simulink model "RobustFormationControl_IntegerModel_under_Dis"  (R2023a)
settings: Solver=ode3  StartTime=0.0  StopTime=30  FixedStep=0.0001  RelTol=1e-3
InitFcn:
  | % % Parameters for the fractional order NTFSMC:
  | % Sliding Surface " Sx, Sy, and Sz ":
  | %------------------------
  | % 10
  | % 10
  | cx = 2*[4 4 4];
  | cxx = 1*[0.01 0.01 0.01];
  | 
  | cx1 = cx(1);
  | cy1 = cx(2);
  | cz1 = cx(3);
  | 
  | cx2 = cxx(1);
  | cy2 = cxx(2);
  | cz2 = cxx(3);
  | 
  | alpha1 = [0.6 0.6 0.6];
  | alpha2 = [0.1 0.1 0.1];
  | 
  | gammaX = [3 3 3];
  | gx  = gammaX(1);
  | gy = gammaX(2);
  | gz = gammaX(3);
  | 
  | p = 10;
  | q = 10;
  | 
  | % Sliding Surface " S_Phi , S_Theta, and  S_Psi":
  | %------------------------
  | cP = 2*[4 4 4];
  | cPP = 1*[0.01 0.01 0.01 0.01];
  | 
  | cPhi1 = cP(1);
  | cTheta1 = cP(2);
  | cPsi1 = cP(3);
  | 
  | cPhi2 = cPP(1);
  | cTheta2 = cPP(2);
  | cPsi2 = cPP(3);
  | gammaP = [3 3 3];
  | 
  | %=========================
  | %=========================
  | SigmaX = 1*[0.01 0.01 0.01];
  | SigmaXX =1*[1 1 1];
  | 
  | Sigma1X = SigmaX(1);
  | Sigma1Y = SigmaX(2);
  | Sigma1Z = SigmaX(3);
  | %-----
  | Sigma2X = SigmaXX(1);
  | Sigma2Y = SigmaXX(2);
  | Sigma2Z = SigmaXX(3);
  | 
  | 
  | SigmaP = 1*[0.01 0.01 0.01];
  | SigmaPP =1*[1 1 1];
  | 
  | Sigma1Phi   = SigmaP(1);
  | Sigma1Theta = SigmaP(2);
  | ... (+80 lines)
values from neighbouring files (symbols this model uses):
  a1 = (Iyy - Izz)/Ixx    (= -0.812397034596)    [init_quadrotor_params.m]
  a2 = (Izz - Ixx)/Iyy    (= 0.812397034596)    [init_quadrotor_params.m]
  a3 = (Ixx - Iyy)/Izz    (= 0)    [init_quadrotor_params.m]
  a4 = - Ktx/m    (= -0.00114547325103)    [init_quadrotor_params.m]
  a5 = - Kty/m    (= -0.00114547325103)    [init_quadrotor_params.m]
  a6 = - Ktz/m    (= -0.00130740740741)    [init_quadrotor_params.m]
  b = 2.980e-5    (= 2.98e-05)    [init_quadrotor_params.m]
  b1 = - Jr/Ixx    (= -0.00584534596376)    [init_quadrotor_params.m]
  b2 = Jr/Iyy    (= 0.00584534596376)    [init_quadrotor_params.m]
  b3 = - Kfz/Izz    (= -0.0721963413248)    [init_quadrotor_params.m]
  b4 = 1/m    (= 2.05761316872)    [init_quadrotor_params.m]
  b5 = 1/m    (= 2.05761316872)    [init_quadrotor_params.m]
  b6 = 1/m    (= 2.05761316872)    [init_quadrotor_params.m]
  c1 = - Kfx/Ixx    (= -0.114641680395)    [init_quadrotor_params.m]
  c2 = - Kfy/Iyy    (= -0.114641680395)    [init_quadrotor_params.m]
  c3 = 1/Izz    (= 113.62345188)    [init_quadrotor_params.m]
  d = 1.12e-06    [init_quadrotor_params.m]
  d1 = L/Ixx    (= 46.334431631)    [init_quadrotor_params.m]
  d2 = L/Iyy    (= 46.334431631)    [init_quadrotor_params.m]
  g = 9.81    [init_quadrotor_params.m]
  Ixx = 4.856e-3    (= 0.004856)    [init_quadrotor_params.m]
  Iyy = 4.856e-3    (= 0.004856)    [init_quadrotor_params.m]
  Izz = 8.801e-3    (= 0.008801)    [init_quadrotor_params.m]
  Jr = 2.8385e-5    (= 2.8385e-05)    [init_quadrotor_params.m]
  Kfx = 5.567e-4    (= 0.0005567)    [init_quadrotor_params.m]
  Kfy = 5.567e-4    (= 0.0005567)    [init_quadrotor_params.m]
  Kfz = 6.354e-4    (= 0.0006354)    [init_quadrotor_params.m]
  Ktx = 5.5670e-4    (= 0.0005567)    [init_quadrotor_params.m]
  Kty = 5.5670e-4    (= 0.0005567)    [init_quadrotor_params.m]
  Ktz = 6.3540e-4    (= 0.0006354)    [init_quadrotor_params.m]
  L = 0.225    [init_quadrotor_params.m]
  m = 0.486    [init_quadrotor_params.m]
libraries: fod x120, eeStairGenerator x5
(part 6 of 9)

== system RobustFormationControl_IntegerModel_under_Dis/Integer Leader and four followers/Follower 1 System/Follower 1 Quadrotor Model/Control Module1/Subsystem5/Subsystem ==
  x5 : Inport
  xd5 : Inport  Port=2
  x6 : Inport  Port=3
  xd6 : Inport  Port=4
  S4 : Inport  Port=5
  Constant : Constant  Value=p/q
  Constant1 : Constant  Value=gammaP(3)-1
  Divide : Product  Inputs=**  RndMeth=Zero  SaturateOnIntegerOverflow=on
  Fractional derivative : fod/Fractional derivative  gam=alpha1(3)  ww=[0.001; 1000]  n=5  nFod=off
      settings: SourceProductName=FOMCON Toolbox
  Fractional integrator1 : fod/Fractional integrator  gam=alpha2(2)  ww=[0.001; 1000]  n=5  nFod=off
      settings: SourceProductName=FOMCON Toolbox
  Gain : Gain  Gain=cPsi1
  Gain1 : Gain  Gain=cPsi2
  Gain2 : Gain  Gain=gammaP(3)
  Gain3 : Gain  Gain=Sigma1Psi
  Gain4 : Gain  Gain=Sigma2Psi
  Power : Math  Operator=pow
  Power1 : Math  Operator=pow
  Sign : Signum
  Sum : Sum
  Sum1 : Sum  Inputs=+-
  Sum2 : Sum  Inputs=---
  Sum3 : Sum  Inputs=+-
  D2 : Outport  VectorParamsAs1DForOutWhenUnconnected=off
  wires:
  xd6/1 -> Sum1/2
  xd5/1 -> Sum3/2
  x5/1 -> Sum3/1
  x6/1 -> Sum1/1
  Sum3/1 -> Power1/1, Power/1
  Constant/1 -> Power/2
  Power/1 -> Gain/1
  Gain/1 -> Fractional derivative/1
  Constant1/1 -> Power1/2
  Power1/1 -> Divide/2
  Divide/1 -> Gain1/1
  Gain1/1 -> Gain2/1
  Sum1/1 -> Divide/1
  Gain2/1 -> Fractional integrator1/1
  S4/1 -> Gain4/1, Sign/1
  Sign/1 -> Gain3/1
  Gain3/1 -> Sum/1
  Gain4/1 -> Sum/2
  Sum/1 -> Sum2/3
  Fractional derivative/1 -> Sum2/1
  Fractional integrator1/1 -> Sum2/2
  Sum2/1 -> D2/1

== system RobustFormationControl_IntegerModel_under_Dis/Integer Leader and four followers/Follower 1 System/Follower 1 Quadrotor Model/Control Module1/Subsystem5/Subsystem1 ==
  x4 : Inport
  x6 : Inport  Port=2
  x2 : Inport  Port=3
  xd6 : Inport  Port=4
  Gain : Gain  Gain=a3
  Gain6 : Gain  Gain=b3
  Math Function : Math  Operator=square  SignedPower=on
  Product1 : Product
  Sum1 : Sum  Inputs=--+
  D1 : Outport
  wires:
  x6/1 -> Math Function/1
  Product1/1 -> Gain/1
  xd6/1 -> Sum1/3
  Gain6/1 -> Sum1/2  "c1 x2^2"
  Math Function/1 -> Gain6/1  "x2^2"
  x2/1 -> Product1/1
  Gain/1 -> Sum1/1  "a1 x4 x6"
  x4/1 -> Product1/2
  Sum1/1 -> D1/1

== system RobustFormationControl_IntegerModel_under_Dis/Integer Leader and four followers/Follower 1 System/Follower 1 Quadrotor Model/Control Module1/Subsystem5/Subsystem2 ==
  x5 : Inport
  xd5 : Inport  Port=2
  x6 : Inport  Port=3
  xd6 : Inport  Port=4
  S6 : Inport  Port=5
  Abs : Abs  SaturateOnIntegerOverflow=off
  Divide{,1..4} (5 alike) : Product  Inputs=**  RndMeth=Zero  SaturateOnIntegerOverflow=on
  Gain : Gain  Gain=q0
  Gain1 : Gain  Gain=q1
  Gain2 : Gain  Gain=q2
  Integrator : Integrator
  Integrator1 : Integrator
  Integrator2 : Integrator
  Sign : Signum
  Sum1 : Sum  Inputs=+-
  Sum2 : Sum  Inputs=----
  Sum3 : Sum  Inputs=+-
  w : Constant  Value=w
  D3 : Outport  VectorParamsAs1DForOutWhenUnconnected=off
  wires:
  xd6/1 -> Sum1/2
  xd5/1 -> Sum3/2
  x5/1 -> Sum3/1
  x6/1 -> Sum1/1
  S6/1 -> [S6], Abs/1
  Sum1/1 -> [e2]
  Sum3/1 -> [e1]
  Gain/1 -> Integrator/1
  Integrator/1 -> Sum2/1  "B0"
  [e1] -> Divide/2
  Gain1/1 -> Integrator1/1
  Divide/1 -> Gain1/1
  Divide1/1 -> Gain2/1
  Gain2/1 -> Integrator2/1
  [e2] -> Divide1/2
  Abs/1 -> Divide1/1, Divide/1, Gain/1
  Integrator1/1 -> Divide3/2  "B1"
  w/1 -> Sum2/4
  Sign/1 -> Divide2/2
  [S6] -> Sign/1
  Divide2/1 -> D3/1
  [e1] -> Divide3/1
  [e2] -> Divide4/1
  Integrator2/1 -> Divide4/2  "B2"
  Divide3/1 -> Sum2/2
  Divide4/1 -> Sum2/3
  Sum2/1 -> Divide2/1

== system RobustFormationControl_IntegerModel_under_Dis/Integer Leader and four followers/Follower 1 System/Follower 1 Quadrotor Model/Control Module1/Subsystem6/Subsystem3 ==
  xL : Inport
  x7 : Inport  Port=2
  x8 : Inport  Port=3
  dX : Inport  Port=4
  S8 : Inport  Port=5
  Constant : Constant  Value=p/q
  Constant1 : Constant  Value=gx-1
  Derivative : Derivative
  Derivative1 : Derivative
  Divide : Product  Inputs=**  RndMeth=Zero  SaturateOnIntegerOverflow=on
  Fractional derivative : fod/Fractional derivative  gam=alpha1(1)  ww=[0.001; 1000]  n=5  nFod=off
      settings: SourceProductName=FOMCON Toolbox
  Fractional integrator1 : fod/Fractional integrator  gam=alpha2(1)  ww=[0.001; 1000]  n=5  nFod=off
      settings: SourceProductName=FOMCON Toolbox
  Gain : Gain  Gain=cx1
  Gain1 : Gain  Gain=cx2
  Gain2 : Gain  Gain=gx
  Gain3 : Gain  Gain=Sigma1X
  Gain4 : Gain  Gain=Sigma2X
  Power : Math  Operator=pow
  Power1 : Math  Operator=pow
  Sign : Signum
  Sum : Sum
  Sum1 : Sum  Inputs=+--
  Sum2 : Sum  Inputs=+++
  Sum3 : Sum  Inputs=+--
  D2 : Outport  VectorParamsAs1DForOutWhenUnconnected=off
  wires:
  Sum3/1 -> Power1/1, Power/1
  Constant/1 -> Power/2
  Power/1 -> Gain/1
  Gain/1 -> Fractional derivative/1
  Constant1/1 -> Power1/2
  Power1/1 -> Divide/2
  Divide/1 -> Gain1/1
  Gain1/1 -> Gain2/1
  Sum1/1 -> Divide/1
  Gain2/1 -> Fractional integrator1/1
  S8/1 -> Gain4/1, Sign/1
  Sign/1 -> Gain3/1
  Gain3/1 -> Sum/1
  Gain4/1 -> Sum/2
  Sum/1 -> Sum2/3
  Fractional derivative/1 -> Sum2/1
  Fractional integrator1/1 -> Sum2/2
  Sum2/1 -> D2/1
  xL/1 -> Sum3/1, Derivative/1
  Derivative/1 -> Sum1/1
  x8/1 -> Sum1/2
  dX/1 -> Sum3/3, Derivative1/1
  Derivative1/1 -> Sum1/3
  x7/1 -> Sum3/2

== system RobustFormationControl_IntegerModel_under_Dis/Integer Leader and four followers/Follower 1 System/Follower 1 Quadrotor Model/Control Module1/Subsystem6/Subsystem4 ==
  x8 : Inport
  xL : Inport  Port=2
  dX : Inport  Port=3
  Derivative{,1..3} (4 alike) : Derivative
  Divide2 : Product  Inputs=**  RndMeth=Zero  SaturateOnIntegerOverflow=on
  Gain1 : Gain  Commented=on  Gain=a6
  Sum : Sum  Inputs=-+-
  D1 : Outport
  wires:
  Sum/1 -> D1/1
  x8/1 -> Divide2/2
  Divide2/1 -> Sum/1
  [a4D] -> Divide2/1
  Derivative/1 -> Derivative1/1
  xL/1 -> Derivative/1
  Derivative3/1 -> Sum/3
  Derivative2/1 -> Derivative3/1
  dX/1 -> Derivative2/1
  Derivative1/1 -> Sum/2

== system RobustFormationControl_IntegerModel_under_Dis/Integer Leader and four followers/Follower 1 System/Follower 1 Quadrotor Model/Control Module1/Subsystem6/Subsystem5 ==
  xL : Inport
  x7 : Inport  Port=2
  x8 : Inport  Port=3
  dX : Inport  Port=4
  S8 : Inport  Port=5
  Abs : Abs  SaturateOnIntegerOverflow=off
  Derivative : Derivative
  Derivative1 : Derivative
  Divide{,1..4} (5 alike) : Product  Inputs=**  RndMeth=Zero  SaturateOnIntegerOverflow=on
  Gain : Gain  Gain=q0
  Gain1 : Gain  Gain=q1
  Gain2 : Gain  Gain=q2
  Integrator : Integrator
  Integrator1 : Integrator
  Integrator2 : Integrator
  Mux : Mux  Inputs=3
  Sign : Signum
  Sum2 : Sum  Inputs=++++
  Sum4 : Sum  Inputs=+--
  Sum5 : Sum  Inputs=+--
  To Workspace : ToWorkspace  VariableName=BxF1  SampleTime=-1
  w : Constant  Value=w
  D3 : Outport  VectorParamsAs1DForOutWhenUnconnected=off
  wires:
  S8/1 -> [S8], Abs/1
  Gain/1 -> Integrator/1
  [e1] -> Divide/2
  Gain1/1 -> Integrator1/1
  Divide/1 -> Gain1/1
  Divide1/1 -> Gain2/1
  Gain2/1 -> Integrator2/1
  [e2] -> Divide1/2
  Abs/1 -> Divide1/1, Divide/1, Gain/1
  Integrator1/1 -> Divide3/2  "B1"
  w/1 -> Sum2/4
  Sign/1 -> Divide2/2
  [S8] -> Sign/1
  Divide2/1 -> D3/1
  [e1] -> Divide3/1
  [e2] -> Divide4/1
  Integrator2/1 -> Divide4/2  "B2"
  Sum2/1 -> Divide2/1
  Derivative1/1 -> Sum4/3
  Derivative/1 -> Sum4/1
  Sum4/1 -> [e2]
  Sum5/1 -> [e1]
  xL/1 -> Sum5/1, Derivative/1
  x8/1 -> Sum4/2
  dX/1 -> Sum5/3, Derivative1/1
  x7/1 -> Sum5/2
  Integrator/1 -> Mux/1, Sum2/1  "B0"
  Divide3/1 -> Mux/2, Sum2/2
  Divide4/1 -> Mux/3, Sum2/3
  Mux/1 -> To Workspace/1

== system RobustFormationControl_IntegerModel_under_Dis/Integer Leader and four followers/Follower 1 System/Follower 1 Quadrotor Model/Control Module1/Subsystem8/Subsystem ==
  x3 : Inport
  xd3 : Inport  Port=2
  x4 : Inport  Port=3
  xd4 : Inport  Port=4
  S4 : Inport  Port=5
  Constant : Constant  Value=p/q
  Constant1 : Constant  Value=gammaP(2)-1
  Divide : Product  Inputs=**  RndMeth=Zero  SaturateOnIntegerOverflow=on
  Fractional derivative : fod/Fractional derivative  gam=alpha1(2)  ww=[0.001; 1000]  n=5  nFod=off
      settings: SourceProductName=FOMCON Toolbox
  Fractional integrator1 : fod/Fractional integrator  gam=alpha2(2)  ww=[0.001; 1000]  n=5  nFod=off
      settings: SourceProductName=FOMCON Toolbox
  Gain : Gain  Gain=cTheta1
  Gain1 : Gain  Gain=cTheta2
  Gain2 : Gain  Gain=gammaP(2)
  Gain3 : Gain  Gain=Sigma1Theta
  Gain4 : Gain  Gain=Sigma2Theta
  Power : Math  Operator=pow
  Power1 : Math  Operator=pow
  Sign : Signum
  Sum : Sum
  Sum1 : Sum  Inputs=+-
  Sum2 : Sum  Inputs=---
  Sum3 : Sum  Inputs=+-
  D2 : Outport  VectorParamsAs1DForOutWhenUnconnected=off
  wires:
  xd4/1 -> Sum1/2
  xd3/1 -> Sum3/2
  x3/1 -> Sum3/1
  x4/1 -> Sum1/1
  Sum3/1 -> Power1/1, Power/1
  Constant/1 -> Power/2
  Power/1 -> Gain/1
  Gain/1 -> Fractional derivative/1
  Constant1/1 -> Power1/2
  Power1/1 -> Divide/2
  Divide/1 -> Gain1/1
  Gain1/1 -> Gain2/1
  Sum1/1 -> Divide/1
  Gain2/1 -> Fractional integrator1/1
  S4/1 -> Gain4/1, Sign/1
  Sign/1 -> Gain3/1
  Gain3/1 -> Sum/1
  Gain4/1 -> Sum/2
  Sum/1 -> Sum2/3
  Fractional derivative/1 -> Sum2/1
  Fractional integrator1/1 -> Sum2/2
  Sum2/1 -> D2/1

== system RobustFormationControl_IntegerModel_under_Dis/Integer Leader and four followers/Follower 1 System/Follower 1 Quadrotor Model/Control Module1/Subsystem8/Subsystem1 ==
  x4 : Inport
  x6 : Inport  Port=2
  x2 : Inport  Port=3
  Omega : Inport  Port=4
  xd4 : Inport  Port=5
  Gain1 : Gain  Gain=a2
  Gain2 : Gain  Gain=c2
  Gain3 : Gain  Gain=b2
  Math Function1 : Math  Operator=square  SignedPower=on
  Product2 : Product
  Product4 : Product
  Sum3 : Sum  Inputs=---+
  D1 : Outport
  wires:
  x6/1 -> Product2/2
  Gain1/1 -> Sum3/1  "a1 x4 x6"
  Sum3/1 -> D1/1
  Math Function1/1 -> Gain2/1  "x2^2"
  x2/1 -> Product4/1, Product2/1
  x4/1 -> Math Function1/1
  xd4/1 -> Sum3/4
  Product4/1 -> Gain3/1
  Omega/1 -> Product4/2
  Product2/1 -> Gain1/1
  Gain3/1 -> Sum3/3
  Gain2/1 -> Sum3/2  "c1 x2^2"

== system RobustFormationControl_IntegerModel_under_Dis/Integer Leader and four followers/Follower 1 System/Follower 1 Quadrotor Model/Control Module1/Subsystem8/Subsystem2 ==
  x3 : Inport
  xd3 : Inport  Port=2
  x4 : Inport  Port=3
  xd4 : Inport  Port=4
  S4 : Inport  Port=5
  Abs : Abs  SaturateOnIntegerOverflow=off
  Divide{,1..4} (5 alike) : Product  Inputs=**  RndMeth=Zero  SaturateOnIntegerOverflow=on
  Gain : Gain  Gain=q0
  Gain1 : Gain  Gain=q1
  Gain2 : Gain  Gain=q2
  Integrator : Integrator
  Integrator1 : Integrator
  Integrator2 : Integrator
  Sign : Signum
  Sum1 : Sum  Inputs=+-
  Sum2 : Sum  Inputs=----
  Sum3 : Sum  Inputs=+-
  w : Constant  Value=w
  D3 : Outport  VectorParamsAs1DForOutWhenUnconnected=off
  wires:
  xd4/1 -> Sum1/2
  xd3/1 -> Sum3/2
  x3/1 -> Sum3/1
  x4/1 -> Sum1/1
  S4/1 -> [S4], Abs/1
  Sum1/1 -> [e2]
  Sum3/1 -> [e1]
  Gain/1 -> Integrator/1
  Integrator/1 -> Sum2/1  "B0"
  [e1] -> Divide/2
  Gain1/1 -> Integrator1/1
  Divide/1 -> Gain1/1
  Divide1/1 -> Gain2/1
  Gain2/1 -> Integrator2/1
  [e2] -> Divide1/2
  Abs/1 -> Divide1/1, Divide/1, Gain/1
  Integrator1/1 -> Divide3/2  "B1"
  w/1 -> Sum2/4
  Sign/1 -> Divide2/2
  [S4] -> Sign/1
  Divide2/1 -> D3/1
  [e1] -> Divide3/1
  [e2] -> Divide4/1
  Integrator2/1 -> Divide4/2  "B2"
  Divide3/1 -> Sum2/2
  Divide4/1 -> Sum2/3
  Sum2/1 -> Divide2/1

== system RobustFormationControl_IntegerModel_under_Dis/Integer Leader and four followers/Follower 1 System/Follower 1 Quadrotor Model/Quadrotor Dynamic System/Rotational System/Equation1 ==
  x4 : Inport
  x6 : Inport  Port=2
  U2 : Inport  Port=3
  Omega : Inport  Port=4
  Gain : Gain  Gain=a1
  Gain1 : Gain  Gain=c1
  Gain2 : Gain  Gain=b1
  Gain3 : Gain  Gain=d1
  Integrator : Integrator
  Integrator1 : Integrator
  Math Function : Math  Operator=square  SignedPower=on
  Product : Product
  Product1 : Product
  Sum : Sum  Inputs=|++++
  x1 = Phi : Outport  VectorParamsAs1DForOutWhenUnconnected=off
  x2 : Outport  Port=2  VectorParamsAs1DForOutWhenUnconnected=off
  wires:
  Math Function/1 -> Gain1/1  "x2^2"
  x4/1 -> Product1/1, Product/1
  Integrator/1 -> Math Function/1, x2/1, Integrator1/1
  U2/1 -> Gain3/1
  Gain2/1 -> Sum/3
  Gain3/1 -> Sum/4
  Gain/1 -> Sum/1  "a1 x4 x6"
  Product1/1 -> Gain2/1
  Gain1/1 -> Sum/2  "c1 x2^2"
  Integrator1/1 -> x1 = Phi/1
  Product/1 -> Gain/1
  x6/1 -> Product/2
  Sum/1 -> Integrator/1
  Omega/1 -> Product1/2

== system RobustFormationControl_IntegerModel_under_Dis/Integer Leader and four followers/Follower 1 System/Follower 1 Quadrotor Model/Quadrotor Dynamic System/Rotational System/Equation2 ==
  x2 : Inport
  x6 : Inport  Port=2
  U3 : Inport  Port=3
  Omega : Inport  Port=4
  Gain : Gain  Gain=a2
  Gain1 : Gain  Gain=c2
  Gain2 : Gain  Gain=b2
  Gain3 : Gain  Gain=d2
  Integrator : Integrator
  Integrator1 : Integrator
  Math Function : Math  Operator=square  SignedPower=on
  Product : Product
  Product1 : Product
  Sum : Sum  Inputs=|++++
  x3 =Theta : Outport  VectorParamsAs1DForOutWhenUnconnected=off
  x4 : Outport  Port=2  VectorParamsAs1DForOutWhenUnconnected=off
  wires:
  Math Function/1 -> Gain1/1  "x4^2"
  x2/1 -> Product1/1, Product/1
  Integrator/1 -> Math Function/1, x4/1, Integrator1/1
  U3/1 -> Gain3/1
  Gain2/1 -> Sum/3
  Gain3/1 -> Sum/4
  Gain/1 -> Sum/1  "a2 x2 x6"
  Product1/1 -> Gain2/1
  Gain1/1 -> Sum/2  "c2 x2^2"
  Integrator1/1 -> x3 =Theta/1
  Product/1 -> Gain/1
  x6/1 -> Product/2
  Sum/1 -> Integrator/1
  Omega/1 -> Product1/2

== system RobustFormationControl_IntegerModel_under_Dis/Integer Leader and four followers/Follower 1 System/Follower 1 Quadrotor Model/Quadrotor Dynamic System/Rotational System/Equation3 ==
  x2 : Inport
  x4 : Inport  Port=2
  U4 : Inport  Port=3
  Gain : Gain  Gain=a3
  Gain1 : Gain  Gain=b3
  Gain3 : Gain  Gain=c3
  Integrator : Integrator
  Integrator1 : Integrator
  Math Function : Math  Operator=square  SignedPower=on
  Product : Product
  Sum : Sum  Inputs=|+++
  x5 =Psi : Outport  VectorParamsAs1DForOutWhenUnconnected=off
  x6 : Outport  Port=2  VectorParamsAs1DForOutWhenUnconnected=off
  wires:
  Math Function/1 -> Gain1/1  "x6^2"
  x2/1 -> Product/1
  Integrator/1 -> Math Function/1, x6/1, Integrator1/1
  U4/1 -> Gain3/1
  Gain3/1 -> Sum/3
  Gain/1 -> Sum/1  "a3 x2 x4"
  Gain1/1 -> Sum/2  "b3 x6^2"
  Integrator1/1 -> x5 =Psi/1
  Product/1 -> Gain/1
  x4/1 -> Product/2
  Sum/1 -> Integrator/1

== system RobustFormationControl_IntegerModel_under_Dis/Integer Leader and four followers/Follower 1 System/Follower 1 Quadrotor Model/Quadrotor Dynamic System/Translational System/Equation4 ==
  U1 : Inport
  Ux : Inport  Port=2
  Gain : Gain  Gain=1/m
  Gain1 : Gain  Gain=a4
  Integrator : Integrator
  Integrator1 : Integrator  InitialCondition=2
  Product : Product
  Sum : Sum  Inputs=|++
  x7 = x : Outport  VectorParamsAs1DForOutWhenUnconnected=off
  x8 = xdot : Outport  Port=2  VectorParamsAs1DForOutWhenUnconnected=off
  wires:
  Integrator/1 -> Gain1/1, x8 = xdot/1, Integrator1/1
  U1/1 -> Product/1
  Gain/1 -> Sum/1  "U1 Ux / m"
  Gain1/1 -> Sum/2  "a4 x8"
  Integrator1/1 -> x7 = x/1
  Product/1 -> Gain/1
  Ux/1 -> Product/2
  Sum/1 -> Integrator/1

== system RobustFormationControl_IntegerModel_under_Dis/Integer Leader and four followers/Follower 1 System/Follower 1 Quadrotor Model/Quadrotor Dynamic System/Translational System/Equation5 ==
  U1 : Inport
  Uy : Inport  Port=2
  Gain : Gain  Gain=1/m
  Gain1 : Gain  Gain=a5
  Integrator : Integrator
  Integrator1 : Integrator  InitialCondition=-2
  Product : Product
  Sum : Sum  Inputs=|++
  x9 = y : Outport  VectorParamsAs1DForOutWhenUnconnected=off
  x10 = ydot : Outport  Port=2  VectorParamsAs1DForOutWhenUnconnected=off
  wires:
  Integrator/1 -> x10 = ydot/1, Integrator1/1, Gain1/1
  U1/1 -> Product/1
  Gain/1 -> Sum/1  "U1 Ux / m"
  Gain1/1 -> Sum/2  "a4 x10"
  Integrator1/1 -> x9 = y/1
  Product/1 -> Gain/1
  Uy/1 -> Product/2
  Sum/1 -> Integrator/1

== system RobustFormationControl_IntegerModel_under_Dis/Integer Leader and four followers/Follower 1 System/Follower 1 Quadrotor Model/Quadrotor Dynamic System/Translational System/Equation6 ==
  U1 : Inport
  x1 : Inport  Port=2
  x3 : Inport  Port=3
  Constant : Constant  Value=g
  Gain : Gain  Gain=1/m
  Gain1 : Gain  Gain=a6
  Integrator : Integrator
  Integrator1 : Integrator
  Product : Product
  Product1 : Product
  Sum : Sum  Inputs=|++-
  Trigonometric Function : Trigonometry  Operator=cos
  Trigonometric Function1 : Trigonometry  Operator=cos
  x11 = z : Outport  VectorParamsAs1DForOutWhenUnconnected=off
  x12 = zdot : Outport  Port=2  VectorParamsAs1DForOutWhenUnconnected=off
  wires:
  U1/1 -> Product/1
  Gain/1 -> Sum/1  "U1 cx1 cx3  / m"
  Gain1/1 -> Sum/2  "a6 x12"
  Integrator1/1 -> x11 = z/1
  Product/1 -> Gain/1
  Sum/1 -> Integrator/1
  Product1/1 -> Product/2
  Trigonometric Function/1 -> Product1/1
  Trigonometric Function1/1 -> Product1/2
  x1/1 -> Trigonometric Function/1
  x3/1 -> Trigonometric Function1/1
  Constant/1 -> Sum/3
  Integrator/1 -> Gain1/1, x12 = zdot/1, Integrator1/1

== system RobustFormationControl_IntegerModel_under_Dis/Integer Leader and four followers/Follower 2 System/Follower 2 Quadrotor Model/Control Module1/Omega Equations/Control Inputs ==
  w1_sqt : Inport
  w2_sqt : Inport  Port=2
  w3_sqt : Inport  Port=3
  w4_sqt : Inport  Port=4
  Add4 : Sum  Inputs=+-+-
  Omega : Outport  VectorParamsAs1DForOutWhenUnconnected=off
  wires:
  Add4/1 -> Omega/1
  w1_sqt/1 -> Add4/1
  w2_sqt/1 -> Add4/2
  w3_sqt/1 -> Add4/3
  w4_sqt/1 -> Add4/4

== system RobustFormationControl_IntegerModel_under_Dis/Integer Leader and four followers/Follower 2 System/Follower 2 Quadrotor Model/Control Module1/Subsystem/Subsystem ==
  Ux : Inport
  Uy : Inport  Port=2
  Psi_d : Inport  Port=3
  Product : Product
  Product1 : Product
  Subtract : Sum  Inputs=+-
  Trigonometric Function : Trigonometry
  Trigonometric Function1 : Trigonometry  Operator=cos
  Trigonometric Function2 : Trigonometry  Operator=asin
  Phi_d : Outport  VectorParamsAs1DForOutWhenUnconnected=off
  wires:
  Product1/1 -> Subtract/2
  Uy/1 -> Product1/2
  Ux/1 -> Product/1
  Trigonometric Function1/1 -> Product1/1
  Psi_d/1 -> Trigonometric Function1/1, Trigonometric Function/1
  Product/1 -> Subtract/1
  Subtract/1 -> Trigonometric Function2/1
  Trigonometric Function/1 -> Product/2
  Trigonometric Function2/1 -> Phi_d/1

== system RobustFormationControl_IntegerModel_under_Dis/Integer Leader and four followers/Follower 2 System/Follower 2 Quadrotor Model/Control Module1/Subsystem/Subsystem1 ==
  Ux : Inport
  Uy : Inport  Port=2
  Psi_d : Inport  Port=3
  Phi_d : Inport  Port=4
  Constant : Constant
  Divide : Product  Inputs=*/
  Product : Product
  Product1 : Product
  Product2 : Product
  Subtract : Sum
  Trigonometric Function : Trigonometry  Operator=cos
  Trigonometric Function1 : Trigonometry
  Trigonometric Function2 : Trigonometry  Operator=asin
  Trigonometric Function3 : Trigonometry  Operator=cos
  Theta_d : Outport  VectorParamsAs1DForOutWhenUnconnected=off
  wires:
  Product1/1 -> Subtract/2
  Uy/1 -> Product1/2
  Ux/1 -> Product/1
  Trigonometric Function1/1 -> Product1/1
  Psi_d/1 -> Trigonometric Function1/1, Trigonometric Function/1
  Product/1 -> Subtract/1
  Trigonometric Function/1 -> Product/2
  Trigonometric Function2/1 -> Theta_d/1
  Constant/1 -> Divide/1
  Product2/1 -> Trigonometric Function2/1
  Subtract/1 -> Product2/1
  Divide/1 -> Product2/2
  Trigonometric Function3/1 -> Divide/2
  Phi_d/1 -> Trigonometric Function3/1

== system RobustFormationControl_IntegerModel_under_Dis/Integer Leader and four followers/Follower 2 System/Follower 2 Quadrotor Model/Control Module1/Subsystem1/Subsystem ==
  x1 : Inport
  xd1 : Inport  Port=2
  x2 : Inport  Port=3
  xd2 : Inport  Port=4
  Constant : Constant  Value=p/q
  Constant1 : Constant  Value=gx
  Divide : Product  Inputs=**  RndMeth=Zero  SaturateOnIntegerOverflow=on
  Fractional integrator : fod/Fractional integrator  gam=alpha1(1)  ww=[0.001; 1000]  n=5  nFod=off
      settings: SourceProductName=FOMCON Toolbox
  Fractional integrator1 : fod/Fractional integrator  gam=alpha2(1)  ww=[0.001; 1000]  n=5  nFod=off
      settings: SourceProductName=FOMCON Toolbox
  Gain : Gain  Gain=cPhi1
  Gain1 : Gain  Gain=cPhi2
  Power : Math  Operator=pow
  Power1 : Math  Operator=pow
  Sign : Signum
  Sum1 : Sum  Inputs=+-
  Sum2 : Sum  Inputs=+++
  Sum3 : Sum  Inputs=+-
  S2 : Outport  VectorParamsAs1DForOutWhenUnconnected=off
  wires:
  xd2/1 -> Sum1/2
  Sum2/1 -> S2/1
  xd1/1 -> Sum3/2
  x1/1 -> Sum3/1
  x2/1 -> Sum1/1
  Sum3/1 -> Power1/1, Sign/1, Power/1
  Constant/1 -> Power/2
  Power/1 -> Gain/1
  Gain/1 -> Fractional integrator/1
  Constant1/1 -> Power1/2
  Sign/1 -> Divide/1
  Power1/1 -> Divide/2
  Divide/1 -> Gain1/1
  Gain1/1 -> Fractional integrator1/1
  Sum1/1 -> Sum2/1
  Fractional integrator/1 -> Sum2/2
  Fractional integrator1/1 -> Sum2/3

== system RobustFormationControl_IntegerModel_under_Dis/Integer Leader and four followers/Follower 2 System/Follower 2 Quadrotor Model/Control Module1/Subsystem1/Subsystem1 ==
  x5 : Inport
  xd5 : Inport  Port=2
  x6 : Inport  Port=3
  xd6 : Inport  Port=4
  Constant : Constant  Value=p/q
  Constant1 : Constant  Value=gz
  Divide : Product  Inputs=**  RndMeth=Zero  SaturateOnIntegerOverflow=on
  Fractional integrator : fod/Fractional integrator  gam=alpha1(3)  ww=[0.001; 1000]  n=5  nFod=off
      settings: SourceProductName=FOMCON Toolbox
  Fractional integrator1 : fod/Fractional integrator  gam=alpha2(3)  ww=[0.001; 1000]  n=5  nFod=off
      settings: SourceProductName=FOMCON Toolbox
  Gain : Gain  Gain=cPsi1
  Gain1 : Gain  Gain=cPsi2
  Power : Math  Operator=pow
  Power1 : Math  Operator=pow
  Sign : Signum
  Sum1 : Sum  Inputs=+-
  Sum2 : Sum  Inputs=+++
  Sum3 : Sum  Inputs=+-
  S6 : Outport  VectorParamsAs1DForOutWhenUnconnected=off
  wires:
  xd6/1 -> Sum1/2
  Sum2/1 -> S6/1
  xd5/1 -> Sum3/2
  x5/1 -> Sum3/1
  x6/1 -> Sum1/1
  Sum3/1 -> Power1/1, Sign/1, Power/1
  Constant/1 -> Power/2
  Power/1 -> Gain/1
  Gain/1 -> Fractional integrator/1
  Constant1/1 -> Power1/2
  Sign/1 -> Divide/1
  Power1/1 -> Divide/2
  Divide/1 -> Gain1/1
  Gain1/1 -> Fractional integrator1/1
  Sum1/1 -> Sum2/1
  Fractional integrator/1 -> Sum2/2
  Fractional integrator1/1 -> Sum2/3

== system RobustFormationControl_IntegerModel_under_Dis/Integer Leader and four followers/Follower 2 System/Follower 2 Quadrotor Model/Control Module1/Subsystem1/Subsystem2 ==
  yL : Inport
  x9 : Inport  Port=2
  x10 : Inport  Port=3
  dY : Inport  Port=4
  Constant : Constant  Value=p/q
  Constant1 : Constant  Value=gy
  Derivative : Derivative
  Derivative1 : Derivative
  Divide : Product  Inputs=**  RndMeth=Zero  SaturateOnIntegerOverflow=on
  Fractional integrator : fod/Fractional integrator  gam=alpha1(2)  ww=[0.001; 1000]  n=5  nFod=off
      settings: SourceProductName=FOMCON Toolbox
  Fractional integrator1 : fod/Fractional integrator  gam=alpha2(2)  ww=[0.001; 1000]  n=5  nFod=off
      settings: SourceProductName=FOMCON Toolbox
  Gain2 : Gain  Gain=cy1
  Gain3 : Gain  Gain=cy2
  Power : Math  Operator=pow
  Power1 : Math  Operator=pow
  Sign : Signum
  Sum1 : Sum  Inputs=+--
  Sum3 : Sum  Inputs=+--
  Sum5 : Sum  Inputs=+++
  S10 : Outport  VectorParamsAs1DForOutWhenUnconnected=off
  wires:
  x9/1 -> Sum3/2
  yL/1 -> Sum3/1, Derivative/1
  dY/1 -> Sum3/3, Derivative1/1
  x10/1 -> Sum1/3
  Derivative/1 -> Sum1/1
  Derivative1/1 -> Sum1/2
  Fractional integrator1/1 -> Sum5/3
  Fractional integrator/1 -> Sum5/2
  Gain3/1 -> Fractional integrator1/1
  Sum1/1 -> Sum5/1
  Sum5/1 -> S10/1
  Divide/1 -> Gain3/1
  Gain2/1 -> Fractional integrator/1
  Sign/1 -> Divide/1
  Power1/1 -> Divide/2
  Power/1 -> Gain2/1
  Constant1/1 -> Power1/2
  Sum3/1 -> Power1/1, Sign/1, Power/1
  Constant/1 -> Power/2

== system RobustFormationControl_IntegerModel_under_Dis/Integer Leader and four followers/Follower 2 System/Follower 2 Quadrotor Model/Control Module1/Subsystem1/Subsystem3 ==
  xL : Inport
  x7 : Inport  Port=2
  x8 : Inport  Port=3
  dX : Inport  Port=4
  Constant : Constant  Value=p/q
  Constant1 : Constant  Value=gx
  Derivative : Derivative
  Derivative1 : Derivative
  Divide : Product  Inputs=**  RndMeth=Zero  SaturateOnIntegerOverflow=on
  Fractional integrator : fod/Fractional integrator  gam=alpha1(1)  ww=[0.001; 1000]  n=5  nFod=off
      settings: SourceProductName=FOMCON Toolbox
  Fractional integrator1 : fod/Fractional integrator  gam=alpha2(1)  ww=[0.001; 1000]  n=5  nFod=off
      settings: SourceProductName=FOMCON Toolbox
  Gain2 : Gain  Gain=cx1
  Gain3 : Gain  Gain=cx2
  Power : Math  Operator=pow
  Power1 : Math  Operator=pow
  Sign : Signum
  Sum1 : Sum  Inputs=+--
  Sum3 : Sum  Inputs=+--
  Sum5 : Sum  Inputs=+++
  S8 : Outport  VectorParamsAs1DForOutWhenUnconnected=off
  wires:
  x7/1 -> Sum3/2
  xL/1 -> Sum3/1, Derivative/1
  dX/1 -> Sum3/3, Derivative1/1
  x8/1 -> Sum1/3
  Derivative/1 -> Sum1/1
  Derivative1/1 -> Sum1/2
  Fractional integrator1/1 -> Sum5/3
  Fractional integrator/1 -> Sum5/2
  Gain3/1 -> Fractional integrator1/1
  Sum1/1 -> Sum5/1
  Sum5/1 -> S8/1
  Divide/1 -> Gain3/1
  Gain2/1 -> Fractional integrator/1
  Sign/1 -> Divide/1
  Power1/1 -> Divide/2
  Power/1 -> Gain2/1
  Constant1/1 -> Power1/2
  Sum3/1 -> Power1/1, Sign/1, Power/1
  Constant/1 -> Power/2

== system RobustFormationControl_IntegerModel_under_Dis/Integer Leader and four followers/Follower 2 System/Follower 2 Quadrotor Model/Control Module1/Subsystem1/Subsystem4 ==
  zL : Inport
  x11 : Inport  Port=2
  x12 : Inport  Port=3
  dZ : Inport  Port=4
  Constant : Constant  Value=p/q
  Constant1 : Constant  Value=gz
  Derivative : Derivative
  Derivative1 : Derivative
  Divide : Product  Inputs=**  RndMeth=Zero  SaturateOnIntegerOverflow=on
  Fractional integrator : fod/Fractional integrator  gam=alpha1(2)  ww=[0.001; 1000]  n=5  nFod=off
      settings: SourceProductName=FOMCON Toolbox
  Fractional integrator1 : fod/Fractional integrator  gam=alpha2(2)  ww=[0.001; 1000]  n=5  nFod=off
      settings: SourceProductName=FOMCON Toolbox
  Gain2 : Gain  Gain=cz1
  Gain3 : Gain  Gain=cz2
  Power : Math  Operator=pow
  Power1 : Math  Operator=pow
  Sign : Signum
  Sum1 : Sum  Inputs=+--
  Sum3 : Sum  Inputs=+--
  Sum5 : Sum  Inputs=+++
  S12 : Outport  VectorParamsAs1DForOutWhenUnconnected=off
  wires:
  Constant/1 -> Power/2
  Sum3/1 -> Power/1, Sign/1, Power1/1
  Constant1/1 -> Power1/2
  Power/1 -> Gain2/1
  Power1/1 -> Divide/2
  Sign/1 -> Divide/1
  Gain2/1 -> Fractional integrator/1
  Divide/1 -> Gain3/1
  Sum5/1 -> S12/1
  Sum1/1 -> Sum5/1
  Gain3/1 -> Fractional integrator1/1
  Fractional integrator/1 -> Sum5/2
  Fractional integrator1/1 -> Sum5/3
  Derivative1/1 -> Sum1/2
  Derivative/1 -> Sum1/1
  x12/1 -> Sum1/3
  dZ/1 -> Derivative1/1, Sum3/3
  zL/1 -> Derivative/1, Sum3/1
  x11/1 -> Sum3/2

== system RobustFormationControl_IntegerModel_under_Dis/Integer Leader and four followers/Follower 2 System/Follower 2 Quadrotor Model/Control Module1/Subsystem1/Subsystem6 ==
  x3 : Inport
  xd3 : Inport  Port=2
  x4 : Inport  Port=3
  xd4 : Inport  Port=4
  Constant : Constant  Value=p/q
  Constant1 : Constant  Value=gy
  Divide : Product  Inputs=**  RndMeth=Zero  SaturateOnIntegerOverflow=on
  Fractional integrator : fod/Fractional integrator  gam=alpha1(2)  ww=[0.001; 1000]  n=5  nFod=off
      settings: SourceProductName=FOMCON Toolbox
  Fractional integrator1 : fod/Fractional integrator  gam=alpha2(2)  ww=[0.001; 1000]  n=5  nFod=off
      settings: SourceProductName=FOMCON Toolbox
  Gain : Gain  Gain=cTheta1
  Gain1 : Gain  Gain=cTheta2
  Power : Math  Operator=pow
  Power1 : Math  Operator=pow
  Sign : Signum
  Sum1 : Sum  Inputs=+-
  Sum2 : Sum  Inputs=+++
  Sum3 : Sum  Inputs=+-
  S4 : Outport  VectorParamsAs1DForOutWhenUnconnected=off
  wires:
  xd4/1 -> Sum1/2
  Sum2/1 -> S4/1
  xd3/1 -> Sum3/2
  x3/1 -> Sum3/1
  x4/1 -> Sum1/1
  Sum3/1 -> Power1/1, Sign/1, Power/1
  Constant/1 -> Power/2
  Power/1 -> Gain/1
  Gain/1 -> Fractional integrator/1
  Constant1/1 -> Power1/2
  Sign/1 -> Divide/1
  Power1/1 -> Divide/2
  Divide/1 -> Gain1/1
  Gain1/1 -> Fractional integrator1/1
  Sum1/1 -> Sum2/1
  Fractional integrator/1 -> Sum2/2
  Fractional integrator1/1 -> Sum2/3

== system RobustFormationControl_IntegerModel_under_Dis/Integer Leader and four followers/Follower 2 System/Follower 2 Quadrotor Model/Control Module1/Subsystem10/Subsystem ==
  zL : Inport
  x11 : Inport  Port=2
  x12 : Inport  Port=3
  dZ : Inport  Port=4
  S12 : Inport  Port=5
  Constant : Constant  Value=p/q
  Constant1 : Constant  Value=gz-1
  Derivative : Derivative
  Derivative1 : Derivative
  Divide : Product  Inputs=**  RndMeth=Zero  SaturateOnIntegerOverflow=on
  Fractional derivative : fod/Fractional derivative  gam=alpha1(3)  ww=[0.001; 1000]  n=5  nFod=off
      settings: SourceProductName=FOMCON Toolbox
  Fractional integrator1 : fod/Fractional integrator  gam=alpha2(3)  ww=[0.001; 1000]  n=5  nFod=off
      settings: SourceProductName=FOMCON Toolbox
  Gain : Gain  Gain=cz1
  Gain1 : Gain  Gain=cz2
  Gain2 : Gain  Gain=gz
  Gain3 : Gain  Gain=Sigma1Z
  Gain4 : Gain  Gain=Sigma2Z
  Power : Math  Operator=pow
  Power1 : Math  Operator=pow
  Sign : Signum
  Sum : Sum
  Sum1 : Sum  Inputs=+--
  Sum2 : Sum  Inputs=+++
  Sum3 : Sum  Inputs=+--
  D2 : Outport  VectorParamsAs1DForOutWhenUnconnected=off
  wires:
  Sum3/1 -> Power1/1, Power/1
  Constant/1 -> Power/2
  Power/1 -> Gain/1
  Gain/1 -> Fractional derivative/1
  Constant1/1 -> Power1/2
  Power1/1 -> Divide/2
  Divide/1 -> Gain1/1
  Gain1/1 -> Gain2/1
  Sum1/1 -> Divide/1
  Gain2/1 -> Fractional integrator1/1
  S12/1 -> Gain4/1, Sign/1
  Sign/1 -> Gain3/1
  Gain3/1 -> Sum/1
  Gain4/1 -> Sum/2
  Sum/1 -> Sum2/3
  Fractional derivative/1 -> Sum2/1
  Fractional integrator1/1 -> Sum2/2
  Sum2/1 -> D2/1
  zL/1 -> Sum3/1, Derivative/1
  Derivative/1 -> Sum1/1
  x12/1 -> Sum1/2
  dZ/1 -> Sum3/3, Derivative1/1
  Derivative1/1 -> Sum1/3
  x11/1 -> Sum3/2

== system RobustFormationControl_IntegerModel_under_Dis/Integer Leader and four followers/Follower 2 System/Follower 2 Quadrotor Model/Control Module1/Subsystem10/Subsystem1 ==
  x12 : Inport
  zL : Inport  Port=2
  dZ : Inport  Port=3
  Constant2 : Constant  Value=g
  Derivative{,1..3} (4 alike) : Derivative
  Divide2 : Product  Inputs=**  RndMeth=Zero  SaturateOnIntegerOverflow=on
  Gain1 : Gain  Commented=on  Gain=a6
  Sum : Sum  Inputs=-++-
  D1 : Outport
  wires:
  Sum/1 -> D1/1
  x12/1 -> Divide2/2
  Divide2/1 -> Sum/1
  Constant2/1 -> Sum/2
  [a6D] -> Divide2/1
  Derivative/1 -> Derivative1/1
  Derivative1/1 -> Sum/3
  zL/1 -> Derivative/1
  Derivative3/1 -> Sum/4
  Derivative2/1 -> Derivative3/1
  dZ/1 -> Derivative2/1

== system RobustFormationControl_IntegerModel_under_Dis/Integer Leader and four followers/Follower 2 System/Follower 2 Quadrotor Model/Control Module1/Subsystem10/Subsystem2 ==
  zL : Inport
  x11 : Inport  Port=2
  x12 : Inport  Port=3
  dZ : Inport  Port=4
  S12 : Inport  Port=5
  Abs : Abs  SaturateOnIntegerOverflow=off
  Derivative : Derivative
  Derivative1 : Derivative
  Divide{,1..4} (5 alike) : Product  Inputs=**  RndMeth=Zero  SaturateOnIntegerOverflow=on
  Gain : Gain  Gain=q0
  Gain1 : Gain  Gain=q1
  Gain2 : Gain  Gain=q2
  Integrator : Integrator
  Integrator1 : Integrator
  Integrator2 : Integrator
  Sign : Signum
  Sum2 : Sum  Inputs=++++
  Sum4 : Sum  Inputs=+--
  Sum5 : Sum  Inputs=+--
  w : Constant  Value=w
  D3 : Outport  VectorParamsAs1DForOutWhenUnconnected=off
  wires:
  S12/1 -> [S12], Abs/1
  Gain/1 -> Integrator/1
  Integrator/1 -> Sum2/1  "B0"
  [e1] -> Divide/2
  Gain1/1 -> Integrator1/1
  Divide/1 -> Gain1/1
  Divide1/1 -> Gain2/1
  Gain2/1 -> Integrator2/1
  [e2] -> Divide1/2
  Abs/1 -> Divide1/1, Divide/1, Gain/1
  Integrator1/1 -> Divide3/2  "B1"
  w/1 -> Sum2/4
  Sign/1 -> Divide2/2
  [S12] -> Sign/1
  Divide2/1 -> D3/1
  [e1] -> Divide3/1
  [e2] -> Divide4/1
  Integrator2/1 -> Divide4/2  "B2"
  Divide3/1 -> Sum2/2
  Divide4/1 -> Sum2/3
  Sum2/1 -> Divide2/1
  Derivative1/1 -> Sum4/3
  Derivative/1 -> Sum4/1
  Sum4/1 -> [e2]
  Sum5/1 -> [e1]
  zL/1 -> Sum5/1, Derivative/1
  x12/1 -> Sum4/2
  dZ/1 -> Sum5/3, Derivative1/1
  x11/1 -> Sum5/2

== system RobustFormationControl_IntegerModel_under_Dis/Integer Leader and four followers/Follower 2 System/Follower 2 Quadrotor Model/Control Module1/Subsystem2/Subsystem3 ==
  yL : Inport
  x9 : Inport  Port=2
  x10 : Inport  Port=3
  dY : Inport  Port=4
  S10 : Inport  Port=5
  Constant : Constant  Value=p/q
  Constant1 : Constant  Value=gy-1
  Derivative : Derivative
  Derivative1 : Derivative
  Divide : Product  Inputs=**  RndMeth=Zero  SaturateOnIntegerOverflow=on
  Fractional derivative : fod/Fractional derivative  gam=alpha1(2)  ww=[0.001; 1000]  n=5  nFod=off
      settings: SourceProductName=FOMCON Toolbox
  Fractional integrator1 : fod/Fractional integrator  gam=alpha2(2)  ww=[0.001; 1000]  n=5  nFod=off
      settings: SourceProductName=FOMCON Toolbox
  Gain : Gain  Gain=cy1
  Gain1 : Gain  Gain=cy2
  Gain2 : Gain  Gain=gy
  Gain3 : Gain  Gain=Sigma1Y
  Gain4 : Gain  Gain=Sigma2Y
  Power : Math  Operator=pow
  Power1 : Math  Operator=pow
  Sign : Signum
  Sum : Sum
  Sum1 : Sum  Inputs=+--
  Sum2 : Sum  Inputs=+++
  Sum3 : Sum  Inputs=+--
  D2 : Outport  VectorParamsAs1DForOutWhenUnconnected=off
  wires:
  Sum3/1 -> Power1/1, Power/1
  Constant/1 -> Power/2
  Power/1 -> Gain/1
  Gain/1 -> Fractional derivative/1
  Constant1/1 -> Power1/2
  Power1/1 -> Divide/2
  Divide/1 -> Gain1/1
  Gain1/1 -> Gain2/1
  Sum1/1 -> Divide/1
  Gain2/1 -> Fractional integrator1/1
  S10/1 -> Gain4/1, Sign/1
  Sign/1 -> Gain3/1
  Gain3/1 -> Sum/1
  Gain4/1 -> Sum/2
  Sum/1 -> Sum2/3
  Fractional derivative/1 -> Sum2/1
  Fractional integrator1/1 -> Sum2/2
  Sum2/1 -> D2/1
  yL/1 -> Sum3/1, Derivative/1
  Derivative/1 -> Sum1/1
  x10/1 -> Sum1/2
  dY/1 -> Sum3/3, Derivative1/1
  Derivative1/1 -> Sum1/3
  x9/1 -> Sum3/2

== system RobustFormationControl_IntegerModel_under_Dis/Integer Leader and four followers/Follower 2 System/Follower 2 Quadrotor Model/Control Module1/Subsystem2/Subsystem4 ==
  x10 : Inport
  yL : Inport  Port=2
  dY : Inport  Port=3
  Derivative{,1..3} (4 alike) : Derivative
  Divide2 : Product  Inputs=**  RndMeth=Zero  SaturateOnIntegerOverflow=on
  Gain1 : Gain  Commented=on  Gain=a5
  Sum : Sum  Inputs=-+-
  D1 : Outport
  wires:
  Sum/1 -> D1/1
  x10/1 -> Divide2/2
  Divide2/1 -> Sum/1
  [a5D] -> Divide2/1
  Derivative/1 -> Derivative1/1
  yL/1 -> Derivative/1
  Derivative3/1 -> Sum/3
  Derivative2/1 -> Derivative3/1
  dY/1 -> Derivative2/1
  Derivative1/1 -> Sum/2

== system RobustFormationControl_IntegerModel_under_Dis/Integer Leader and four followers/Follower 2 System/Follower 2 Quadrotor Model/Control Module1/Subsystem2/Subsystem5 ==
  yL : Inport
  x9 : Inport  Port=2
  x10 : Inport  Port=3
  dY : Inport  Port=4
  S10 : Inport  Port=5
  Abs : Abs  SaturateOnIntegerOverflow=off
  Derivative : Derivative
  Derivative1 : Derivative
  Divide{,1..4} (5 alike) : Product  Inputs=**  RndMeth=Zero  SaturateOnIntegerOverflow=on
  Gain : Gain  Gain=q0
  Gain1 : Gain  Gain=q1
  Gain2 : Gain  Gain=q2
  Integrator : Integrator
  Integrator1 : Integrator
  Integrator2 : Integrator
  Sign : Signum
  Sum2 : Sum  Inputs=++++
  Sum4 : Sum  Inputs=+--
  Sum5 : Sum  Inputs=+--
  w : Constant  Value=w
  D3 : Outport  VectorParamsAs1DForOutWhenUnconnected=off
  wires:
  S10/1 -> [S10], Abs/1
  Gain/1 -> Integrator/1
  Integrator/1 -> Sum2/1  "B0"
  [e1] -> Divide/2
  Gain1/1 -> Integrator1/1
  Divide/1 -> Gain1/1
  Divide1/1 -> Gain2/1
  Gain2/1 -> Integrator2/1
  [e2] -> Divide1/2
  Abs/1 -> Divide1/1, Divide/1, Gain/1
  Integrator1/1 -> Divide3/2  "B1"
  w/1 -> Sum2/4
  Sign/1 -> Divide2/2
  [S10] -> Sign/1
  Divide2/1 -> D3/1
  [e1] -> Divide3/1
  [e2] -> Divide4/1
  Integrator2/1 -> Divide4/2  "B2"
  Divide3/1 -> Sum2/2
  Divide4/1 -> Sum2/3
  Sum2/1 -> Divide2/1
  Derivative1/1 -> Sum4/3
  Derivative/1 -> Sum4/1
  Sum4/1 -> [e2]
  Sum5/1 -> [e1]
  yL/1 -> Sum5/1, Derivative/1
  x10/1 -> Sum4/2
  dY/1 -> Sum5/3, Derivative1/1
  x9/1 -> Sum5/2

== system RobustFormationControl_IntegerModel_under_Dis/Integer Leader and four followers/Follower 2 System/Follower 2 Quadrotor Model/Control Module1/Subsystem4/Subsystem ==
  x1 : Inport
  xd1 : Inport  Port=2
  x2 : Inport  Port=3
  xd2 : Inport  Port=4
  S2 : Inport  Port=5
  Constant : Constant  Value=p/q
  Constant1 : Constant  Value=gammaP(1)-1
  Divide : Product  Inputs=**  RndMeth=Zero  SaturateOnIntegerOverflow=on
  Fractional derivative : fod/Fractional derivative  gam=alpha1(1)  ww=[0.001; 1000]  n=5  nFod=off
      settings: SourceProductName=FOMCON Toolbox
  Fractional integrator1 : fod/Fractional integrator  gam=alpha2(2)  ww=[0.001; 1000]  n=5  nFod=off
      settings: SourceProductName=FOMCON Toolbox
  Gain : Gain  Gain=cPhi1
  Gain1 : Gain  Gain=cPhi2
  Gain2 : Gain  Gain=gammaP(1)
  Gain3 : Gain  Gain=Sigma1Phi
  Gain4 : Gain  Gain=Sigma1Phi
  Power : Math  Operator=pow
  Power1 : Math  Operator=pow
  Sign : Signum
  Sum : Sum
  Sum1 : Sum  Inputs=+-
  Sum2 : Sum  Inputs=---
  Sum3 : Sum  Inputs=+-
  D2 : Outport  VectorParamsAs1DForOutWhenUnconnected=off
  wires:
  xd2/1 -> Sum1/2
  xd1/1 -> Sum3/2
  x1/1 -> Sum3/1
  x2/1 -> Sum1/1
  Sum3/1 -> Power1/1, Power/1
  Constant/1 -> Power/2
  Power/1 -> Gain/1
  Gain/1 -> Fractional derivative/1
  Constant1/1 -> Power1/2
  Power1/1 -> Divide/2
  Divide/1 -> Gain1/1
  Gain1/1 -> Gain2/1
  Sum1/1 -> Divide/1
  Gain2/1 -> Fractional integrator1/1
  S2/1 -> Gain4/1, Sign/1
  Sign/1 -> Gain3/1
  Gain3/1 -> Sum/1
  Gain4/1 -> Sum/2
  Sum/1 -> Sum2/3
  Fractional derivative/1 -> Sum2/1
  Fractional integrator1/1 -> Sum2/2
  Sum2/1 -> D2/1

== system RobustFormationControl_IntegerModel_under_Dis/Integer Leader and four followers/Follower 2 System/Follower 2 Quadrotor Model/Control Module1/Subsystem4/Subsystem1 ==
  x4 : Inport
  x6 : Inport  Port=2
  x2 : Inport  Port=3
  Omega : Inport  Port=4
  xd2 : Inport  Port=5
  Gain : Gain  Gain=a1
  Gain6 : Gain  Gain=c1
  Gain7 : Gain  Gain=b1
  Math Function : Math  Operator=square  SignedPower=on
  Product1 : Product
  Product3 : Product
  Sum3 : Sum  Inputs=---+
  D1 : Outport
  wires:
  xd2/1 -> Sum3/4
  Product1/1 -> Gain/1
  Sum3/1 -> D1/1
  Gain6/1 -> Sum3/2  "c1 x2^2"
  Gain7/1 -> Sum3/3
  Product3/1 -> Gain7/1
  Omega/1 -> Product3/2
  Math Function/1 -> Gain6/1  "x2^2"
  x4/1 -> Product3/1, Product1/1
  Gain/1 -> Sum3/1  "a1 x4 x6"
  x6/1 -> Product1/2
  x2/1 -> Math Function/1

== system RobustFormationControl_IntegerModel_under_Dis/Integer Leader and four followers/Follower 2 System/Follower 2 Quadrotor Model/Control Module1/Subsystem4/Subsystem2 ==
  x1 : Inport
  xd1 : Inport  Port=2
  x2 : Inport  Port=3
  xd2 : Inport  Port=4
  S2 : Inport  Port=5
  Abs : Abs  SaturateOnIntegerOverflow=off
  Divide{,1..4} (5 alike) : Product  Inputs=**  RndMeth=Zero  SaturateOnIntegerOverflow=on
  Gain : Gain  Gain=q0
  Gain1 : Gain  Gain=q1
  Gain2 : Gain  Gain=q2
  Integrator : Integrator
  Integrator1 : Integrator
  Integrator2 : Integrator
  Sign : Signum
  Sum1 : Sum  Inputs=+-
  Sum2 : Sum  Inputs=----
  Sum3 : Sum  Inputs=+-
  w : Constant  Value=w
  D3 : Outport  VectorParamsAs1DForOutWhenUnconnected=off
  wires:
  xd2/1 -> Sum1/2
  xd1/1 -> Sum3/2
  x1/1 -> Sum3/1
  x2/1 -> Sum1/1
  S2/1 -> [S2], Abs/1
  Sum1/1 -> [e2]
  Sum3/1 -> [e1]
  Gain/1 -> Integrator/1
  Integrator/1 -> Sum2/1  "B0"
  [e1] -> Divide/2
  Gain1/1 -> Integrator1/1
  Divide/1 -> Gain1/1
  Divide1/1 -> Gain2/1
  Gain2/1 -> Integrator2/1
  [e2] -> Divide1/2
  Abs/1 -> Divide1/1, Divide/1, Gain/1
  Integrator1/1 -> Divide3/2  "B1"
  w/1 -> Sum2/4
  Sign/1 -> Divide2/2
  [S2] -> Sign/1
  Divide2/1 -> D3/1
  [e1] -> Divide3/1
  [e2] -> Divide4/1
  Integrator2/1 -> Divide4/2  "B2"
  Divide3/1 -> Sum2/2
  Divide4/1 -> Sum2/3
  Sum2/1 -> Divide2/1

== system RobustFormationControl_IntegerModel_under_Dis/Integer Leader and four followers/Follower 2 System/Follower 2 Quadrotor Model/Control Module1/Subsystem5/Subsystem ==
  x5 : Inport
  xd5 : Inport  Port=2
  x6 : Inport  Port=3
  xd6 : Inport  Port=4
  S4 : Inport  Port=5
  Constant : Constant  Value=p/q
  Constant1 : Constant  Value=gammaP(3)-1
  Divide : Product  Inputs=**  RndMeth=Zero  SaturateOnIntegerOverflow=on
  Fractional derivative : fod/Fractional derivative  gam=alpha1(3)  ww=[0.001; 1000]  n=5  nFod=off
      settings: SourceProductName=FOMCON Toolbox
  Fractional integrator1 : fod/Fractional integrator  gam=alpha2(2)  ww=[0.001; 1000]  n=5  nFod=off
      settings: SourceProductName=FOMCON Toolbox
  Gain : Gain  Gain=cPsi1
  Gain1 : Gain  Gain=cPsi2
  Gain2 : Gain  Gain=gammaP(3)
  Gain3 : Gain  Gain=Sigma1Psi
  Gain4 : Gain  Gain=Sigma2Psi
  Power : Math  Operator=pow
  Power1 : Math  Operator=pow
  Sign : Signum
  Sum : Sum
  Sum1 : Sum  Inputs=+-
  Sum2 : Sum  Inputs=---
  Sum3 : Sum  Inputs=+-
  D2 : Outport  VectorParamsAs1DForOutWhenUnconnected=off
  wires:
  xd6/1 -> Sum1/2
  xd5/1 -> Sum3/2
  x5/1 -> Sum3/1
  x6/1 -> Sum1/1
  Sum3/1 -> Power1/1, Power/1
  Constant/1 -> Power/2
  Power/1 -> Gain/1
  Gain/1 -> Fractional derivative/1
  Constant1/1 -> Power1/2
  Power1/1 -> Divide/2
  Divide/1 -> Gain1/1
  Gain1/1 -> Gain2/1
  Sum1/1 -> Divide/1
  Gain2/1 -> Fractional integrator1/1
  S4/1 -> Gain4/1, Sign/1
  Sign/1 -> Gain3/1
  Gain3/1 -> Sum/1
  Gain4/1 -> Sum/2
  Sum/1 -> Sum2/3
  Fractional derivative/1 -> Sum2/1
  Fractional integrator1/1 -> Sum2/2
  Sum2/1 -> D2/1

== system RobustFormationControl_IntegerModel_under_Dis/Integer Leader and four followers/Follower 2 System/Follower 2 Quadrotor Model/Control Module1/Subsystem5/Subsystem1 ==
  x4 : Inport
  x6 : Inport  Port=2
  x2 : Inport  Port=3
  xd6 : Inport  Port=4
  Gain : Gain  Gain=a3
  Gain6 : Gain  Gain=b3
  Math Function : Math  Operator=square  SignedPower=on
  Product1 : Product
  Sum1 : Sum  Inputs=--+
  D1 : Outport
  wires:
  x6/1 -> Math Function/1
  Product1/1 -> Gain/1
  xd6/1 -> Sum1/3
  Gain6/1 -> Sum1/2  "c1 x2^2"
  Math Function/1 -> Gain6/1  "x2^2"
  x2/1 -> Product1/1
  Gain/1 -> Sum1/1  "a1 x4 x6"
  x4/1 -> Product1/2
  Sum1/1 -> D1/1

== system RobustFormationControl_IntegerModel_under_Dis/Integer Leader and four followers/Follower 2 System/Follower 2 Quadrotor Model/Control Module1/Subsystem5/Subsystem2 ==
  x5 : Inport
  xd5 : Inport  Port=2
  x6 : Inport  Port=3
  xd6 : Inport  Port=4
  S6 : Inport  Port=5
  Abs : Abs  SaturateOnIntegerOverflow=off
  Divide{,1..4} (5 alike) : Product  Inputs=**  RndMeth=Zero  SaturateOnIntegerOverflow=on
  Gain : Gain  Gain=q0
  Gain1 : Gain  Gain=q1
  Gain2 : Gain  Gain=q2
  Integrator : Integrator
  Integrator1 : Integrator
  Integrator2 : Integrator
  Sign : Signum
  Sum1 : Sum  Inputs=+-
  Sum2 : Sum  Inputs=----
  Sum3 : Sum  Inputs=+-
  w : Constant  Value=w
  D3 : Outport  VectorParamsAs1DForOutWhenUnconnected=off
  wires:
  xd6/1 -> Sum1/2
  xd5/1 -> Sum3/2
  x5/1 -> Sum3/1
  x6/1 -> Sum1/1
  S6/1 -> [S6], Abs/1
  Sum1/1 -> [e2]
  Sum3/1 -> [e1]
  Gain/1 -> Integrator/1
  Integrator/1 -> Sum2/1  "B0"
  [e1] -> Divide/2
  Gain1/1 -> Integrator1/1
  Divide/1 -> Gain1/1
  Divide1/1 -> Gain2/1
  Gain2/1 -> Integrator2/1
  [e2] -> Divide1/2
  Abs/1 -> Divide1/1, Divide/1, Gain/1
  Integrator1/1 -> Divide3/2  "B1"
  w/1 -> Sum2/4
  Sign/1 -> Divide2/2
  [S6] -> Sign/1
  Divide2/1 -> D3/1
  [e1] -> Divide3/1
  [e2] -> Divide4/1
  Integrator2/1 -> Divide4/2  "B2"
  Divide3/1 -> Sum2/2
  Divide4/1 -> Sum2/3
  Sum2/1 -> Divide2/1

== system RobustFormationControl_IntegerModel_under_Dis/Integer Leader and four followers/Follower 2 System/Follower 2 Quadrotor Model/Control Module1/Subsystem6/Subsystem3 ==
  xL : Inport
  x7 : Inport  Port=2
  x8 : Inport  Port=3
  dX : Inport  Port=4
  S8 : Inport  Port=5
  Constant : Constant  Value=p/q
  Constant1 : Constant  Value=gx-1
  Derivative : Derivative
  Derivative1 : Derivative
  Divide : Product  Inputs=**  RndMeth=Zero  SaturateOnIntegerOverflow=on
  Fractional derivative : fod/Fractional derivative  gam=alpha1(1)  ww=[0.001; 1000]  n=5  nFod=off
      settings: SourceProductName=FOMCON Toolbox
  Fractional integrator1 : fod/Fractional integrator  gam=alpha2(1)  ww=[0.001; 1000]  n=5  nFod=off
      settings: SourceProductName=FOMCON Toolbox
  Gain : Gain  Gain=cx1
  Gain1 : Gain  Gain=cx2
  Gain2 : Gain  Gain=gx
  Gain3 : Gain  Gain=Sigma1X
  Gain4 : Gain  Gain=Sigma2X
  Power : Math  Operator=pow
  Power1 : Math  Operator=pow
  Sign : Signum
  Sum : Sum
  Sum1 : Sum  Inputs=+--
  Sum2 : Sum  Inputs=+++
  Sum3 : Sum  Inputs=+--
  D2 : Outport  VectorParamsAs1DForOutWhenUnconnected=off
  wires:
  Sum3/1 -> Power1/1, Power/1
  Constant/1 -> Power/2
  Power/1 -> Gain/1
  Gain/1 -> Fractional derivative/1
  Constant1/1 -> Power1/2
  Power1/1 -> Divide/2
  Divide/1 -> Gain1/1
  Gain1/1 -> Gain2/1
  Sum1/1 -> Divide/1
  Gain2/1 -> Fractional integrator1/1
  S8/1 -> Gain4/1, Sign/1
  Sign/1 -> Gain3/1
  Gain3/1 -> Sum/1
  Gain4/1 -> Sum/2
  Sum/1 -> Sum2/3
  Fractional derivative/1 -> Sum2/1
  Fractional integrator1/1 -> Sum2/2
  Sum2/1 -> D2/1
  xL/1 -> Sum3/1, Derivative/1
  Derivative/1 -> Sum1/1
  x8/1 -> Sum1/2
  dX/1 -> Sum3/3, Derivative1/1
  Derivative1/1 -> Sum1/3
  x7/1 -> Sum3/2

== system RobustFormationControl_IntegerModel_under_Dis/Integer Leader and four followers/Follower 2 System/Follower 2 Quadrotor Model/Control Module1/Subsystem6/Subsystem4 ==
  x8 : Inport
  xL : Inport  Port=2
  dX : Inport  Port=3
  Derivative{,1..3} (4 alike) : Derivative
  Divide2 : Product  Inputs=**  RndMeth=Zero  SaturateOnIntegerOverflow=on
  Gain1 : Gain  Commented=on  Gain=a6
  Sum : Sum  Inputs=-+-
  D1 : Outport
  wires:
  Sum/1 -> D1/1
  x8/1 -> Divide2/2
  Divide2/1 -> Sum/1
  [a4D] -> Divide2/1
  Derivative/1 -> Derivative1/1
  xL/1 -> Derivative/1
  Derivative3/1 -> Sum/3
  Derivative2/1 -> Derivative3/1
  dX/1 -> Derivative2/1
  Derivative1/1 -> Sum/2
